simulink model "g3p_set_goal"  (R2019b)
settings: Solver=FixedStepAuto  StartTime=0.0  StopTime=10.0  RelTol=1e-3
libraries: robotlib x2
settings Model: Creator=Boen  LastModifiedBy=Boen
settings OptimizationCC: EnhancedBackFolding=on  PassReuseOutputArgsAs=Individual arguments  ZeroExternalMemoryAtStartup=off  ZeroInternalMemoryAtStartup=off  MaxStackSize=64  OptimizeBlockOrder=speed  DifferentSizesBufferReuse=on  OptimizationCustomize=off  EfficientTunableParamExpr=on
settings DebuggingCC: ParameterTunabilityLossMsg=error
settings HardwareCC: ProdBitPerPointer=32  ProdBitPerSizeT=32  ProdBitPerPtrDiffT=32  ProdLargestAtomicInteger=Long  ProdWordSize=32  ProdHWDeviceType=ARM Compatible->ARM 8
settings SFSimCC: MATLABDynamicMemAlloc=off
settings RTWCC: SystemTargetFile=ert.tlc  HardwareBoard=Robot Operating System (ROS)  TLCOptions="-aInlineSetEventsForThisBaseRateFcn=TLC_FALSE -aSuppressMultiTaskScheduler=TLC_FALSE  -aRateBasedStepFcn=0"  TemplateMakefile=ert_default_tmf  GenerateReport=on  Toolchain=Catkin  IncludeHyperlinkInReport=on  LaunchReport=on  TargetLang=C++  GenerateTraceInfo=on  GenerateTraceReport=on  GenerateTraceReportSl=on  GenerateTraceReportSf=on  GenerateTraceReportEml=on
settings CodeAppCC: ForceParamTrailComments=on  IgnoreCustomStorageClasses=off  OperatorAnnotations=on  SimulinkDataObjDesc=on  SFDataObjDesc=on  InsertBlockDesc=on

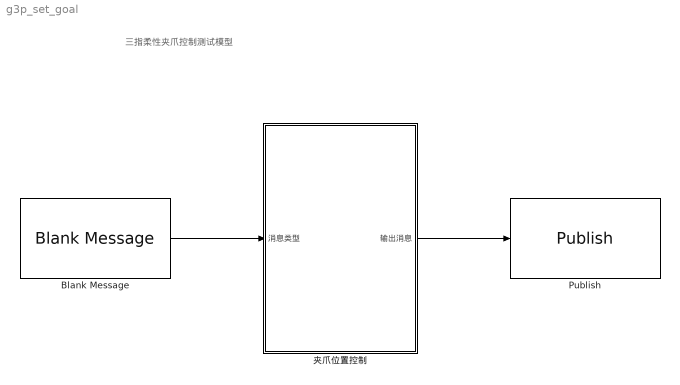
== system g3p_set_goal ==
  note: 三指柔性夹爪控制测试模型
  Blank Message : robotlib/Blank Message  messageClass=Message  entityType=g3p_msgs/Gripper  messageType=g3p_msgs/Gripper  SampleTime=inf
      settings: SourceProductName=ROS Toolbox
  Publish : robotlib/Publish  topicSource=Specify your own  topic=/g3p_msgs/gripper  messageType=g3p_msgs/Gripper  messageQueueLength=1
      settings: SourceProductName=ROS Toolbox
  夹爪位置控制 : Subsystem  mask{MOTOR_STEP=0}
      mask DialogControl DescGroupVar Prompt: 电机行程控制
      mask DialogControl DescTextVar Prompt: 行程范围0cm~11cm
      mask DialogControl ParameterGroupVar Prompt: 输入行程
  wires:
  Blank Message/1 -> 夹爪位置控制/1(消息类型)
  夹爪位置控制/1(输出消息) -> Publish/1

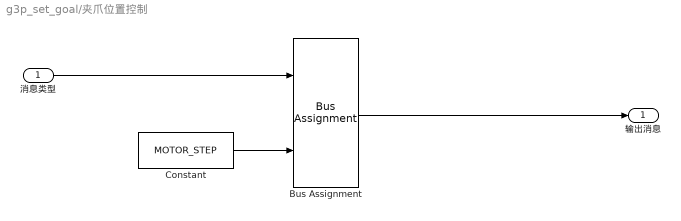
== system g3p_set_goal/夹爪位置控制 ==
  消息类型 : Inport
  Bus Assignment : BusAssignment  AssignedSignals=State
  Constant : Constant  Value=MOTOR_STEP  OutDataTypeStr=double
  输出消息 : Outport
  wires:
  Bus Assignment/1 -> 输出消息/1
  Constant/1 -> Bus Assignment/2
  消息类型/1 -> Bus Assignment/1
